simulink library "Teleop_lib"  (R2023b)
settings: Solver=VariableStepAuto  StartTime=0.0  StopTime=10.0  RelTol=1e-3
undefined symbols (not defined in the file): Spline_Num_Poses_default, Spline_Ref_Poses_default, TEST_Swerve_Mode_Override_Flag, TEST_Swerve_Mode_Steering, TEST_Swerve_Mode_Translation
settings Model: Creator=FIRSTMentor  LastModifiedBy=ander

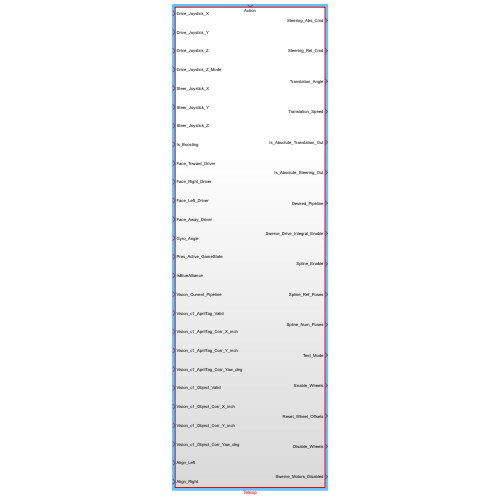
[thumbnail: Simulink's stored preview of the top-level diagram]
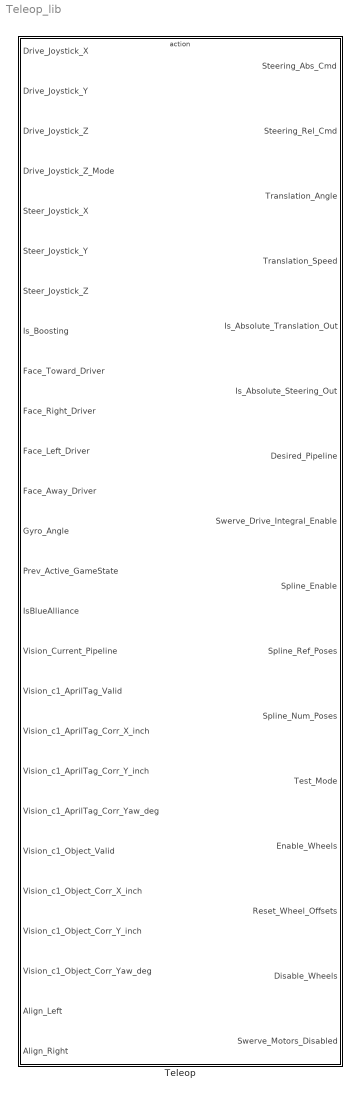
== system Teleop_lib ==
  Teleop : Subsystem  TreatAsAtomicUnit=on

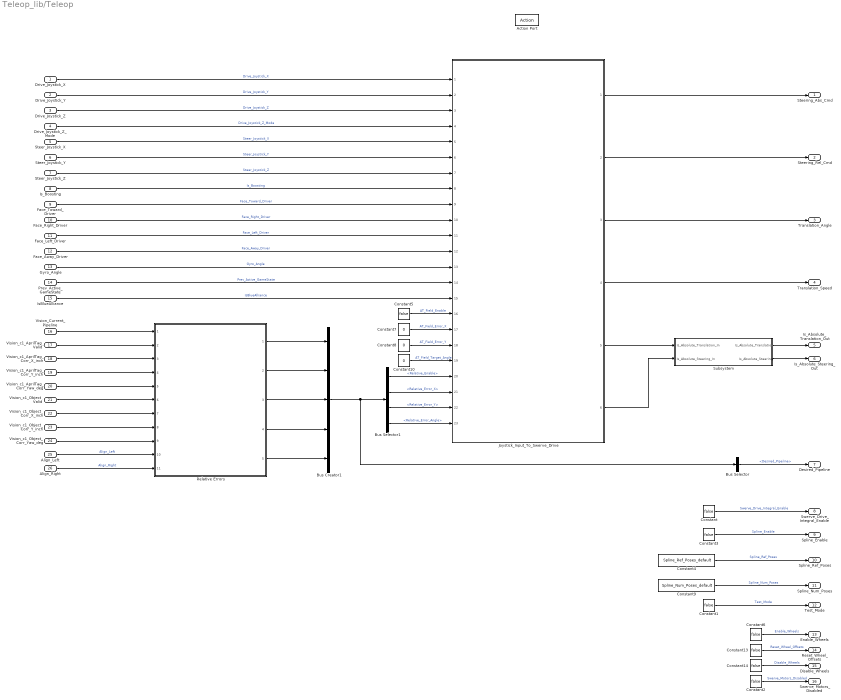
== system Teleop_lib/Teleop ==
  Drive_Joystick_X : Inport
  Drive_Joystick_Y : Inport  Port=2
  Drive_Joystick_Z : Inport  Port=3
  Drive_Joystick_Z_Mode : Inport  Port=4
  Steer_Joystick_X : Inport  Port=5
  Steer_Joystick_Y : Inport  Port=6
  Steer_Joystick_Z : Inport  Port=7
  Is_Boosting : Inport  Port=8
  Face_Toward_Driver : Inport  Port=9
  Face_Right_Driver : Inport  Port=10
  Face_Left_Driver : Inport  Port=11
  Face_Away_Driver : Inport  Port=12
  Gyro_Angle : Inport  Port=13
  Prev_Active_GameState : Inport  Port=14
  IsBlueAlliance : Inport  Port=15
  Vision_Current_Pipeline : Inport  Port=16
  Vision_c1_AprilTag_Valid : Inport  Port=17
  Vision_c1_AprilTag_Corr_X_inch : Inport  Port=18
  Vision_c1_AprilTag_Corr_Y_inch : Inport  Port=19
  Vision_c1_AprilTag_Corr_Yaw_deg : Inport  Port=20
  Vision_c1_Object_Valid : Inport  Port=21
  Vision_c1_Object_Corr_X_inch : Inport  Port=22
  Vision_c1_Object_Corr_Y_inch : Inport  Port=23
  Vision_c1_Object_Corr_Yaw_deg : Inport  Port=24
  Align_Left : Inport  Port=25
  Align_Right : Inport  Port=26
  Action Port : ActionPort  InitializeStates=reset
  Bus Creator1 : BusCreator  Inputs=5
  Bus Selector : BusSelector  OutputSignals=Desired_Pipeline
  Bus Selector1 : BusSelector  OutputSignals=Relative_Enable,Relative_Error_X,Relative_Error_Y,Relative_Error_Angle
  Constant{,1..3,5..6,13..14} (8 alike) : Constant  Value=false  OutDataTypeStr=boolean
  Constant10 : Constant  Value=0
  Constant4 : Constant  Value=Spline_Ref_Poses_default
  Constant7 : Constant  Value=0
  Constant8 : Constant  Value=0
  Constant9 : Constant  Value=Spline_Num_Poses_default  OutDataTypeStr=double
  Joystick_Input_To_Swerve_Drive : Subsystem  ReferencedSubsystem=Joystick_Input_To_Swerve_Drive_sub
  Relative Errors : Subsystem  ReferencedSubsystem=Vision_Relative_Errors_sub
  Subsystem : Subsystem
  Steering_Abs_Cmd : Outport
  Steering_Rel_Cmd : Outport  Port=2
  Translation_Angle : Outport  Port=3
  Translation_Speed : Outport  Port=4
  Is_Absolute_Translation_Out : Outport  Port=5
  Is_Absolute_Steering_Out : Outport  Port=6
  Desired_Pipeline : Outport  Port=7
  Swerve_Drive_Integral_Enable : Outport  Port=8
  Spline_Enable : Outport  Port=9
  Spline_Ref_Poses : Outport  Port=10
  Spline_Num_Poses : Outport  Port=11
  Test_Mode : Outport  Port=12
  Enable_Wheels : Outport  Port=13
  Reset_Wheel_Offsets : Outport  Port=14
  Disable_Wheels : Outport  Port=15
  Swerve_Motors_Disabled : Outport  Port=16
  wires:
  Vision_c1_Object_Valid/1 -> Relative Errors/6
  Vision_c1_AprilTag_Valid/1 -> Relative Errors/2
  Vision_c1_Object_Corr_Yaw_deg/1 -> Relative Errors/9
  Vision_c1_Object_Corr_Y_inch/1 -> Relative Errors/8
  Vision_c1_Object_Corr_X_inch/1 -> Relative Errors/7
  Constant/1 -> Swerve_Drive_Integral_Enable/1  "Swerve_Drive_Integral_Enable"
  Steer_Joystick_X/1 -> Joystick_Input_To_Swerve_Drive/5  "Steer_Joystick_X"
  Steer_Joystick_Y/1 -> Joystick_Input_To_Swerve_Drive/6  "Steer_Joystick_Y"
  Drive_Joystick_X/1 -> Joystick_Input_To_Swerve_Drive/1  "Drive_Joystick_X"
  Drive_Joystick_Y/1 -> Joystick_Input_To_Swerve_Drive/2  "Drive_Joystick_Y"
  Joystick_Input_To_Swerve_Drive/1 -> Steering_Abs_Cmd/1
  Joystick_Input_To_Swerve_Drive/2 -> Steering_Rel_Cmd/1
  Joystick_Input_To_Swerve_Drive/3 -> Translation_Angle/1
  Joystick_Input_To_Swerve_Drive/4 -> Translation_Speed/1
  Is_Boosting/1 -> Joystick_Input_To_Swerve_Drive/8  "Is_Boosting"
  Constant9/1 -> Spline_Num_Poses/1  "Spline_Num_Poses"
  Constant4/1 -> Spline_Ref_Poses/1  "Spline_Ref_Poses"
  Constant3/1 -> Spline_Enable/1  "Spline_Enable"
  Constant1/1 -> Test_Mode/1  "Test_Mode"
  Drive_Joystick_Z/1 -> Joystick_Input_To_Swerve_Drive/3  "Drive_Joystick_Z"
  Steer_Joystick_Z/1 -> Joystick_Input_To_Swerve_Drive/7  "Steer_Joystick_Z"
  Face_Toward_Driver/1 -> Joystick_Input_To_Swerve_Drive/9  "Face_Toward_Driver"
  Face_Right_Driver/1 -> Joystick_Input_To_Swerve_Drive/10  "Face_Right_Driver"
  Face_Left_Driver/1 -> Joystick_Input_To_Swerve_Drive/11  "Face_Left_Driver"
  Face_Away_Driver/1 -> Joystick_Input_To_Swerve_Drive/12  "Face_Away_Driver"
  IsBlueAlliance/1 -> Joystick_Input_To_Swerve_Drive/15  "IsBlueAlliance"
  Drive_Joystick_Z_Mode/1 -> Joystick_Input_To_Swerve_Drive/4  "Drive_Joystick_Z_Mode"
  Gyro_Angle/1 -> Joystick_Input_To_Swerve_Drive/13  "Gyro_Angle"
  Constant13/1 -> Reset_Wheel_Offsets/1  "Reset_Wheel_Offsets"
  Constant14/1 -> Disable_Wheels/1  "Disable_Wheels"
  Prev_Active_GameState/1 -> Joystick_Input_To_Swerve_Drive/14  "Prev_Active_GameState"
  Constant2/1 -> Swerve_Motors_Disabled/1  "Swerve_Motors_Disabled"
  Constant6/1 -> Enable_Wheels/1  "Enable_Wheels"
  Joystick_Input_To_Swerve_Drive/5 -> Subsystem/1(Is_Absolute_Translation_In)
  Joystick_Input_To_Swerve_Drive/6 -> Subsystem/2(Is_Absolute_Steering_In)
  Subsystem/1(Is_Absolute_Translation) -> Is_Absolute_Translation_Out/1
  Subsystem/2(Is_Absolute_Steering) -> Is_Absolute_Steering_Out/1
  Bus Creator1/1 -> Bus Selector1/1, Bus Selector/1
  Bus Selector1/1 -> Joystick_Input_To_Swerve_Drive/20  "<Relative_Enable>"
  Bus Selector1/2 -> Joystick_Input_To_Swerve_Drive/21  "<Relative_Error_X>"
  Bus Selector1/3 -> Joystick_Input_To_Swerve_Drive/22  "<Relative_Error_Y>"
  Bus Selector1/4 -> Joystick_Input_To_Swerve_Drive/23  "<Relative_Error_Angle>"
  Constant5/1 -> Joystick_Input_To_Swerve_Drive/16  "AT_Field_Enable"
  Constant7/1 -> Joystick_Input_To_Swerve_Drive/17  "AT_Field_Error_X"
  Constant8/1 -> Joystick_Input_To_Swerve_Drive/18  "AT_Field_Error_Y"
  Constant10/1 -> Joystick_Input_To_Swerve_Drive/19  "AT_Field_Target_Angle"
  Align_Left/1 -> Relative Errors/10  "Align_Left"
  Align_Right/1 -> Relative Errors/11  "Align_Right"
  Relative Errors/1 -> Bus Creator1/1
  Relative Errors/2 -> Bus Creator1/2
  Relative Errors/3 -> Bus Creator1/3
  Relative Errors/4 -> Bus Creator1/4
  Relative Errors/5 -> Bus Creator1/5
  Bus Selector/1 -> Desired_Pipeline/1  "<Desired_Pipeline>"
  Vision_Current_Pipeline/1 -> Relative Errors/1
  Vision_c1_AprilTag_Corr_X_inch/1 -> Relative Errors/3
  Vision_c1_AprilTag_Corr_Y_inch/1 -> Relative Errors/4
  Vision_c1_AprilTag_Corr_Yaw_deg/1 -> Relative Errors/5

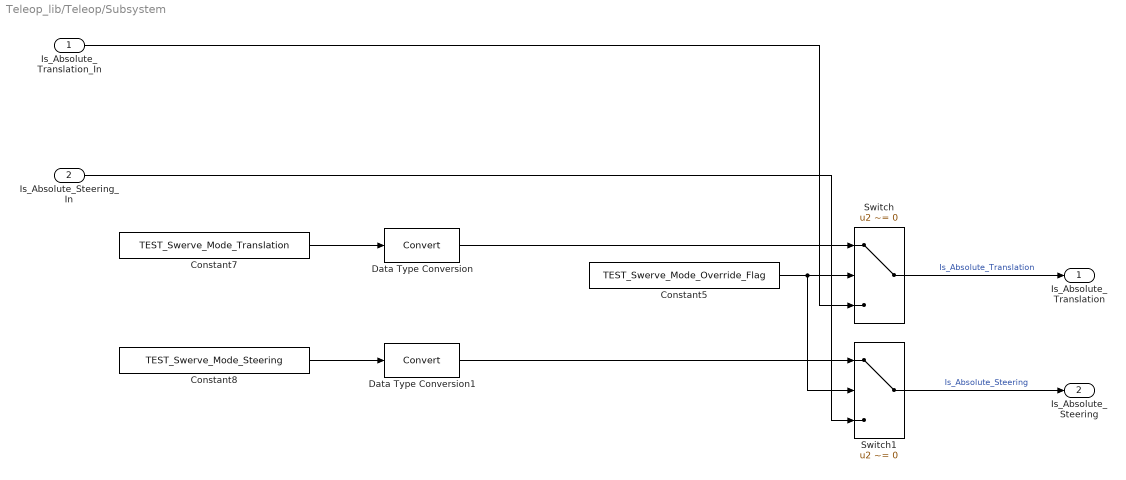
== system Teleop_lib/Teleop/Subsystem ==
  Is_Absolute_Translation_In : Inport
  Is_Absolute_Steering_In : Inport  Port=2
  Constant5 : Constant  Value=TEST_Swerve_Mode_Override_Flag
  Constant7 : Constant  Value=TEST_Swerve_Mode_Translation
  Constant8 : Constant  Value=TEST_Swerve_Mode_Steering
  Data Type Conversion : DataTypeConversion  SaturateOnIntegerOverflow=off  RndMeth=Floor
  Data Type Conversion1 : DataTypeConversion  SaturateOnIntegerOverflow=off  RndMeth=Floor
  Switch : Switch  Criteria=u2 ~= 0  SaturateOnIntegerOverflow=off  InputSameDT=off
  Switch1 : Switch  Criteria=u2 ~= 0  SaturateOnIntegerOverflow=off  InputSameDT=off
  Is_Absolute_Translation : Outport
  Is_Absolute_Steering : Outport  Port=2
  wires:
  Constant5/1 -> Switch/2, Switch1/2
  Data Type Conversion/1 -> Switch/1
  Data Type Conversion1/1 -> Switch1/1
  Is_Absolute_Translation_In/1 -> Switch/3
  Switch/1 -> Is_Absolute_Translation/1  "Is_Absolute_Translation"
  Constant8/1 -> Data Type Conversion1/1
  Constant7/1 -> Data Type Conversion/1
  Is_Absolute_Steering_In/1 -> Switch1/3
  Switch1/1 -> Is_Absolute_Steering/1  "Is_Absolute_Steering"
